simulink model "Crazyflie_Simulation_WSKim"  (R2026b)
settings: Solver=ode15s  StopTime=20  RelTol=1e-5
InitFcn:
  | Crazyflie_Param
values from neighbouring files (symbols this model uses):
  g = 9.80665    [Crazyflie_Param.m]
  Ix_drone = 2.934e-5    (= 2.934e-05)    [Crazyflie_Param.m]
  Iy_drone = 4.981e-5    (= 4.981e-05)    [Crazyflie_Param.m]
  Iz_drone = 7.646e-5    (= 7.646e-05)    [Crazyflie_Param.m]
  J = 1/12*m*(0.051^2+0.005^2)    (= 7.878e-08)    [Crazyflie_Param.m]
  l1 = 4.445    [Crazyflie_Param.m]
  m = 0.00036    [Crazyflie_Param.m]
  m_drone = 0.04316    [Crazyflie_Param.m]
undefined symbols (not defined in the file or in its folder): sigbuilder_block, X, Y, Z
libraries: sm_lib x52, slpidlib x19, nesl_utility x18, fl_lib x5
(part 4 of 4)

== system Crazyflie_Simulation_WSKim/quadrotor model/Rotor4 ==
  "  Motor Thrust 4" : sm_lib/Forces and Torques/External Force and Torque  EnableForceX=off  EnableForceY=off  EnableForceZ=on  EnableForce=off  ForceResolutionFrame=AttachedFrame  EnableTorqueX=off  EnableTorqueY=off  EnableTorqueZ=off  EnableTorque=off  TorqueResolutionFrame=AttachedFrame
  Revolute Joint4 : sm_lib/Joints/Revolute Joint  JointMode=Normal  CompositeWrenchDir=FollowerOnBase  CompositeWrenchFrame=BaseFrame  SenseConstraintForce=off  SenseConstraintTorque=off  SenseTotalForce=off  SenseTotalTorque=off  PositionTargetSpecify=off  PositionTargetPriority=High  PositionTargetValue=0  PositionTargetValueUnits=deg  VelocityTargetSpecify=off  VelocityTargetPriority=High  VelocityTargetValue=0  VelocityTargetValueUnits=deg/s  EquilibriumPosition=0  EquilibriumPositionUnits=rad  SpringStiffness=0  SpringStiffnessUnits=N*m/rad  DampingCoefficient=b  DampingCoefficientUnits=N*m/(rad/s)  LowerLimitSpecify=off  LowerLimitBound=-90  LowerLimitBoundUnits=deg  LowerLimitStiffness=1e4  LowerLimitStiffnessUnits=N*m/deg  LowerLimitDamping=10  LowerLimitDampingUnits=N*m/(deg/s)  LowerLimitTransitionRegionWidth=0.1  LowerLimitTransitionRegionWidthUnits=deg  UpperLimitSpecify=off  UpperLimitBound=90  UpperLimitBoundUnits=deg  UpperLimitStiffness=1e4  UpperLimitStiffnessUnits=N*m/deg  UpperLimitDamping=10  UpperLimitDampingUnits=N*m/(deg/s)  UpperLimitTransitionRegionWidth=0.1  UpperLimitTransitionRegionWidthUnits=deg  TorqueActuationMode=ComputedTorque  MotionActuationMode=InputMotion  SensePosition=off  SenseVelocity=off  SenseAcceleration=off  SenseTorqueForce=off  SenseLowerLimitTorqueForce=off  SenseUpperLimitTorqueForce=off
  Rigid Transform13 : sm_lib/Frames and Transforms/Rigid Transform  RotationMethod=None  FollAlignAxisA=+X  BaseAlignAxisA=+Y  FollAlignAxisB=+Y  BaseAlignAxisB=+Z  RotationStandardAxis=+Z  RotationAngle=0.0  RotationAngleUnits=deg  RotationArbitraryAxis=[0 0 1]  RotationSequenceAxes=FollowerAxes  RotationSequence=XYX  RotationSequenceAngles=[0 0 0]  RotationSequenceAnglesUnits=deg  RotationMatrix=[1 0 0; 0 1 0; 0 0 1]  Quaternion=[1 0 0 0]  TranslationMethod=Cartesian  TranslationCartesianOffset=[0 0 -0.2]  TranslationCartesianOffsetUnits=cm  TranslationStandardAxis=+Z  TranslationStandardOffset=0  TranslationStandardOffsetUnits=cm  TranslationROffset=0  TranslationROffsetUnits=m  TranslationThetaOffset=0  TranslationThetaOffsetUnits=deg  TranslationZOffset=0  TranslationZOffsetUnits=m
  Rigid Transform3 : sm_lib/Frames and Transforms/Rigid Transform  RotationMethod=None  FollAlignAxisA=+X  BaseAlignAxisA=+Y  FollAlignAxisB=+Y  BaseAlignAxisB=+Z  RotationStandardAxis=+Z  RotationAngle=0.0  RotationAngleUnits=deg  RotationArbitraryAxis=[0 0 1]  RotationSequenceAxes=FollowerAxes  RotationSequence=XYX  RotationSequenceAngles=[0 0 0]  RotationSequenceAnglesUnits=deg  RotationMatrix=[1 0 0; 0 1 0; 0 0 1]  Quaternion=[1 0 0 0]  TranslationMethod=Cartesian  TranslationCartesianOffset=[0 -l1 0]  TranslationCartesianOffsetUnits=cm  TranslationStandardAxis=+Z  TranslationStandardOffset=0  TranslationStandardOffsetUnits=cm  TranslationROffset=0  TranslationROffsetUnits=m  TranslationThetaOffset=0  TranslationThetaOffsetUnits=deg  TranslationZOffset=0  TranslationZOffsetUnits=m
  Rigid Transform9 : sm_lib/Frames and Transforms/Rigid Transform  RotationMethod=None  FollAlignAxisA=+X  BaseAlignAxisA=+Y  FollAlignAxisB=+Y  BaseAlignAxisB=+Z  RotationStandardAxis=+Z  RotationAngle=0.0  RotationAngleUnits=deg  RotationArbitraryAxis=[0 0 1]  RotationSequenceAxes=FollowerAxes  RotationSequence=XYX  RotationSequenceAngles=[0 0 0]  RotationSequenceAnglesUnits=deg  RotationMatrix=[1 0 0; 0 1 0; 0 0 1]  Quaternion=[1 0 0 0]  TranslationMethod=Cartesian  TranslationCartesianOffset=[0 0 -1.4]  TranslationCartesianOffsetUnits=cm  TranslationStandardAxis=+Z  TranslationStandardOffset=0  TranslationStandardOffsetUnits=cm  TranslationROffset=0  TranslationROffsetUnits=m  TranslationThetaOffset=0  TranslationThetaOffsetUnits=deg  TranslationZOffset=0  TranslationZOffsetUnits=m
  motor 4 : sm_lib/Body Elements/Cylindrical Solid  CylinderRadius=0.35  CylinderRadiusUnits=cm  CylinderLength=1.7  CylinderLengthUnits=cm  ExportEntireGeometry=off  InertiaType=PointMass  BasedOnType=Density  Density=1000  DensityUnits=kg/m^3  Mass=0  MassUnits=g  CenterOfMass=[0 0 0]  CenterOfMassUnits=m  MomentsOfInertia=[1 1 1]  MomentsOfInertiaUnits=kg*m^2  ProductsOfInertia=[1 1 1]  ProductsOfInertiaUnits=kg*m^2  GraphicType=FromGeometry  MarkerShape=Sphere  MarkerSize=10  GraphicVisPropType=SimpleVisualProperties  GraphicDiffuseColor=[0.4 0.4 0.4]  GraphicOpacity=1.0  GraphicSpecularColor=[0.5 0.5 0.5 1.0]  GraphicAmbientColor=[0.15 0.15 0.15 1.0]  GraphicEmissiveColor=[0.0 0.0 0.0 1.0]  GraphicShininess=75  DoExposeReferenceFrame=on  SerializedFrames=<Frames/>
  rotor4 : sm_lib/Body Elements/Brick Solid  BrickDimensions=[5 0.5 0.1]  BrickDimensionsUnits=cm  ExportEntireGeometry=off  InertiaType=Custom  BasedOnType=Density  Density=1000  DensityUnits=kg/m^3  Mass=m  MassUnits=kg  CenterOfMass=[0 0 0]  CenterOfMassUnits=m  MomentsOfInertia=[0 0 J]  MomentsOfInertiaUnits=kg*m^2  ProductsOfInertia=[0 0 0]  ProductsOfInertiaUnits=kg*m^2  GraphicType=FromGeometry  MarkerShape=Sphere  MarkerSize=10  GraphicVisPropType=SimpleVisualProperties  GraphicDiffuseColor=[1.0 1.0 1.0]  GraphicOpacity=1.0  GraphicSpecularColor=[0.5 0.5 0.5 1.0]  GraphicAmbientColor=[0.15 0.15 0.15 1.0]  GraphicEmissiveColor=[0.0 0.0 0.0 1.0]  GraphicShininess=75  DoExposeReferenceFrame=on  SerializedFrames=<Frames/>
  Revolute Joint : PMIOPort  Side=Right
  Thrust : PMIOPort  Port=2  Side=Right
  Body : PMIOPort  Port=3  Side=Left
  connections:
  Rigid Transform9/LConn1 -- Rigid Transform13/LConn1 -- Rigid Transform3/RConn1
  motor 4/RConn1 -- Rigid Transform13/RConn1
  Revolute Joint4/RConn1 -- rotor4/RConn1
  "  Motor Thrust 4"/RConn1 -- Revolute Joint4/LConn1 -- Rigid Transform9/RConn1
  Revolute Joint/RConn1 -- Revolute Joint4/LConn2
  Body/RConn1 -- Rigid Transform3/LConn1
  Thrust/RConn1 -- "  Motor Thrust 4"/LConn1

== system Crazyflie_Simulation_WSKim/quadrotor model/Thrust and Roatation3 ==
  PWM : Inport
  Integrator2 : Integrator
  Simulink-PS Converter4 : nesl_utility/Simulink-PS Converter  PhysicalDomain=network_engine_domain  SubClassName=ps_input  LeftPortType=input  RightPortType=output  PseudoPeriodic=off  Frequencies=[]  NoiseDistribution=none  NoiseParameters=[]  Unit=1  AffineConversion=off  FilteringAndDerivatives=provide  SimscapeFilterOrder=1  InputFilterTimeConstant=0.001  UdotUserProvided=0
  Simulink-PS Converter5 : nesl_utility/Simulink-PS Converter  PhysicalDomain=network_engine_domain  SubClassName=ps_input  LeftPortType=input  RightPortType=output  PseudoPeriodic=off  Frequencies=[]  NoiseDistribution=none  NoiseParameters=[]  Unit=1  AffineConversion=off  FilteringAndDerivatives=filter  SimscapeFilterOrder=2  InputFilterTimeConstant=0.001  UdotUserProvided=0
  pwm to thrust2 : Fcn  Expr=-(2.130295*10^(-11)*u^2 + 1.032633*10^(-6)*u + 5.484560*10^(-4))
  pwm to w2 : Fcn  Expr=(0.03950236*u + 420.9420)*(u>1000)
  Rotation : PMIOPort  Side=Right
  Thrust : PMIOPort  Port=2  Side=Right
  wires:
  PWM/1 -> pwm to thrust2/1, pwm to w2/1
  pwm to thrust2/1 -> Simulink-PS Converter4/1
  pwm to w2/1 -> Integrator2/1  "dth"
  Integrator2/1 -> Simulink-PS Converter5/1
  connections:
  Simulink-PS Converter4/RConn1 -- Thrust/RConn1
  Simulink-PS Converter5/RConn1 -- Rotation/RConn1

== system Crazyflie_Simulation_WSKim/quadrotor model/Thrust and Rotation1 ==
  PWM : Inport
  Integrator : Integrator
  Simulink-PS Converter1 : nesl_utility/Simulink-PS Converter  PhysicalDomain=network_engine_domain  SubClassName=ps_input  LeftPortType=input  RightPortType=output  PseudoPeriodic=off  Frequencies=[]  NoiseDistribution=none  NoiseParameters=[]  Unit=1  AffineConversion=off  FilteringAndDerivatives=provide  SimscapeFilterOrder=1  InputFilterTimeConstant=0.001  UdotUserProvided=0
  Simulink-PS Converter9 : nesl_utility/Simulink-PS Converter  PhysicalDomain=network_engine_domain  SubClassName=ps_input  LeftPortType=input  RightPortType=output  PseudoPeriodic=off  Frequencies=[]  NoiseDistribution=none  NoiseParameters=[]  Unit=1  AffineConversion=off  FilteringAndDerivatives=filter  SimscapeFilterOrder=2  InputFilterTimeConstant=0.001  UdotUserProvided=0
  pwm to thrust : Fcn  Expr=-(2.130295*10^(-11)*u^2 + 1.032633*10^(-6)*u + 5.484560*10^(-4))
  pwm to w : Fcn  Expr=(0.03950236*u + 420.9420)*(u>1000)
  Rotation : PMIOPort  Side=Right
  Thrust : PMIOPort  Port=2  Side=Right
  wires:
  Integrator/1 -> Simulink-PS Converter9/1  "th"
  pwm to w/1 -> Integrator/1  "dth"
  pwm to thrust/1 -> Simulink-PS Converter1/1
  PWM/1 -> pwm to w/1, pwm to thrust/1
  connections:
  Simulink-PS Converter9/RConn1 -- Rotation/RConn1
  Simulink-PS Converter1/RConn1 -- Thrust/RConn1

== system Crazyflie_Simulation_WSKim/quadrotor model/Thrust and Rotation2 ==
  PWM : Inport
  Gain2 : Gain  Gain=-1
  Integrator1 : Integrator
  Simulink-PS Converter2 : nesl_utility/Simulink-PS Converter  PhysicalDomain=network_engine_domain  SubClassName=ps_input  LeftPortType=input  RightPortType=output  PseudoPeriodic=off  Frequencies=[]  NoiseDistribution=none  NoiseParameters=[]  Unit=1  AffineConversion=off  FilteringAndDerivatives=provide  SimscapeFilterOrder=1  InputFilterTimeConstant=0.001  UdotUserProvided=0
  Simulink-PS Converter3 : nesl_utility/Simulink-PS Converter  PhysicalDomain=network_engine_domain  SubClassName=ps_input  LeftPortType=input  RightPortType=output  PseudoPeriodic=off  Frequencies=[]  NoiseDistribution=none  NoiseParameters=[]  Unit=1  AffineConversion=off  FilteringAndDerivatives=filter  SimscapeFilterOrder=2  InputFilterTimeConstant=0.001  UdotUserProvided=0
  pwm to thrust1 : Fcn  Expr=-(2.130295*10^(-11)*u^2 + 1.032633*10^(-6)*u + 5.484560*10^(-4))
  pwm to w1 : Fcn  Expr=(0.03950236*u + 420.9420)*(u>1000)
  Rotation : PMIOPort  Side=Right
  Thrust : PMIOPort  Port=2  Side=Right
  wires:
  pwm to thrust1/1 -> Simulink-PS Converter2/1
  pwm to w1/1 -> Integrator1/1  "dth"
  Gain2/1 -> Simulink-PS Converter3/1  "th"
  PWM/1 -> pwm to w1/1, pwm to thrust1/1
  Integrator1/1 -> Gain2/1  "th"
  connections:
  Simulink-PS Converter3/RConn1 -- Rotation/RConn1
  Simulink-PS Converter2/RConn1 -- Thrust/RConn1

== system Crazyflie_Simulation_WSKim/quadrotor model/Thrust and Rotation4 ==
  PWM : Inport
  Gain4 : Gain  Gain=-1
  Integrator3 : Integrator
  Simulink-PS Converter6 : nesl_utility/Simulink-PS Converter  PhysicalDomain=network_engine_domain  SubClassName=ps_input  LeftPortType=input  RightPortType=output  PseudoPeriodic=off  Frequencies=[]  NoiseDistribution=none  NoiseParameters=[]  Unit=1  AffineConversion=off  FilteringAndDerivatives=provide  SimscapeFilterOrder=1  InputFilterTimeConstant=0.001  UdotUserProvided=0
  Simulink-PS Converter7 : nesl_utility/Simulink-PS Converter  PhysicalDomain=network_engine_domain  SubClassName=ps_input  LeftPortType=input  RightPortType=output  PseudoPeriodic=off  Frequencies=[]  NoiseDistribution=none  NoiseParameters=[]  Unit=1  AffineConversion=off  FilteringAndDerivatives=filter  SimscapeFilterOrder=2  InputFilterTimeConstant=0.001  UdotUserProvided=0
  pwm to thrust3 : Fcn  Expr=-(2.130295*10^(-11)*u^2 + 1.032633*10^(-6)*u + 5.484560*10^(-4))
  pwm to w3 : Fcn  Expr=(0.03950236*u + 420.9420)*(u>1000)
  Rotation : PMIOPort  Side=Right
  Thrust : PMIOPort  Port=2  Side=Right
  wires:
  pwm to thrust3/1 -> Simulink-PS Converter6/1
  Integrator3/1 -> Gain4/1  "th"
  PWM/1 -> pwm to thrust3/1, pwm to w3/1
  pwm to w3/1 -> Integrator3/1  "dth"
  Gain4/1 -> Simulink-PS Converter7/1  "th"
  connections:
  Simulink-PS Converter6/RConn1 -- Thrust/RConn1
  Simulink-PS Converter7/RConn1 -- Rotation/RConn1

== system Crazyflie_Simulation_WSKim/6dof joint/x,y,z joint/Ground Contact ==
  Ground Contact : Subsystem
  Mechanical Translational Reference : fl_lib/Mechanical/Translational Elements/Mechanical Translational Reference
  Translational Hard Stop : fl_lib/Mechanical/Translational Elements/Translational Hard Stop  upper_bnd=10 m  lower_bnd=0 m  model=3  stiff_up=1e6 N/m  stiff_low=1e6 N/m  D_up=150 N/(m/s)  D_low=150 N/(m/s)  transition=0.1 mm  coeff_rest=0.7  v_tol=0.001 m/s  f_tol=0.001 N  v_specify=off  v_priority=None  v=0 m/s  v_nominal_specify=off  v_nominal_value=1  v_nominal_unit=m/s  f_specify=off  f_priority=None  f=0 N  f_nominal_specify=off  f_nominal_value=1  f_nominal_unit=N  x_specify=off  x_priority=High  x=0 m  x_nominal_specify=off  x_nominal_value=1  x_nominal_unit=m  M_specify=off  M_priority=None  M=0
  Conn1 : PMIOPort  Side=Left
  Conn2 : PMIOPort  Port=2  Side=Right
  connections:
  Conn2/RConn1 -- Ground Contact/RConn1
  Mechanical Translational Reference/LConn1 -- Ground Contact/RConn2 -- Translational Hard Stop/LConn1
  Conn1/RConn1 -- Ground Contact/LConn1
  Ground Contact/LConn2 -- Translational Hard Stop/RConn1

== system Crazyflie_Simulation_WSKim/6dof joint/x,y,z joint/Ground Contact/Ground Contact ==
  Ideal Force Sensor : fl_lib/Mechanical/Mechanical Sensors/Ideal Force Sensor
  Ideal Translational Velocity Source : fl_lib/Mechanical/Mechanical Sources/Ideal Translational Velocity Source
  V : PMIOPort  Side=Right
  F : PMIOPort  Port=2  Side=Left
  C : PMIOPort  Port=3  Side=Left
  R : PMIOPort  Port=4  Side=Right
  connections:
  F/RConn1 -- Ideal Force Sensor/RConn2
  V/RConn1 -- Ideal Translational Velocity Source/RConn1
  Ideal Force Sensor/LConn1 -- Ideal Translational Velocity Source/RConn2
  R/RConn1 -- Ideal Translational Velocity Source/LConn1
  Ideal Force Sensor/RConn1 -- C/RConn1
